simulink model "s_b4a4x32kf_nb"  (R2018a)
settings: Solver=VariableStepDiscrete  StartTime=0.0  StopTime=10000  RelTol=1e-3
undefined symbols (not defined in the file): fft_stages, n_bits_ants, n_bits_xengs
libraries: xbsIndex_r4 x21193, casper_library_misc x37, casper_library_scopes x13, casper_library_delays x8, xbsReplacements_r4 x6, xps_library x4
(part 162 of 274)

== system s_b4a4x32kf_nb/sys2/vacc/hmc_vacc/fifo_rd_cnt ==
  out_reg : Inport
  assert_reg : xbsIndex_r4/Assert  assert_type=on  type_source=Explicitly  gui_display_data_type=Fixed-point  arith_type=Unsigned  n_bits=32  bin_pt=0  preci_type=Single  exp_width=8  frac_width=24  assert_rate=off  rate_source=Explicitly  period=1  output_port=on  block_type=assert
      settings: SourceProductName=The database /home/jmanley/.matlab/R2018a/slblocks_master.db is locked, or a table in the database is locked. (database is locked)
  cast_gw : xbsIndex_r4/Convert  gui_display_data_type=Fixed-point  arith_type=Unsigned  n_bits=32  bin_pt=0  float_type=Single  exp_bits=8  fraction_bits=24  quantization=Truncate  overflow=Wrap  en=off  latency=1  pipeline=off  dbl_ovrd=off  block_type=convert
      settings: SourceProductName=The database /home/jmanley/.matlab/R2018a/slblocks_master.db is locked, or a table in the database is locked. (database is locked)
  io_delay : xbsIndex_r4/Delay  rst=off  infoeditControl=Selection of Reset will increase slice count due to use of real FFs and instead of SRLs  en=off  latency=0  reg_retiming=on  dbl_ovrd=off  block_type=delay
      settings: SourceProductName=The database /home/jmanley/.matlab/R2018a/slblocks_master.db is locked, or a table in the database is locked. (database is locked)
  reint1 : xbsIndex_r4/Reinterpret  force_arith_type=on  arith_type=Unsigned  force_bin_pt=on  bin_pt=0  block_type=reinterpret
      settings: SourceProductName=The database /home/jmanley/.matlab/R2018a/slblocks_master.db is locked, or a table in the database is locked. (database is locked)
  s_b4a4x32kf_nb_sys2_vacc_hmc_vacc_fifo_rd_cnt_user_data_in : xbsIndex_r4/Gateway Out  inherit_from_input=off  hdl_port=on  rows=1  columns=1  UseAsDAC=off  DACChannel='1'  interface=None  automatic_assignment=on  address_offset=hex2dec('00')  intf_name=''  intf_description=''  timing_constraint=None  locs_specified=off  LOCs={}  io_standard={}  block_type=gatewayout
      settings: SourceProductName=The database /home/jmanley/.matlab/R2018a/slblocks_master.db is locked, or a table in the database is locked. (database is locked)
  sim_out : Terminator
  wires:
  io_delay/1 -> cast_gw/1
  cast_gw/1 -> s_b4a4x32kf_nb_sys2_vacc_hmc_vacc_fifo_rd_cnt_user_data_in/1
  s_b4a4x32kf_nb_sys2_vacc_hmc_vacc_fifo_rd_cnt_user_data_in/1 -> sim_out/1
  out_reg/1 -> assert_reg/1
  assert_reg/1 -> reint1/1
  reint1/1 -> io_delay/1

== system s_b4a4x32kf_nb/sys2/vacc/hmc_vacc/fifo_status ==
  out_fetch_valid : Inport
  out_fetch_empty : Inport  Port=2
  out_fetch_full : Inport  Port=3
  out_fetch_afull : Inport  Port=4
  out_rst : Inport  Port=5
  out_fifo_rd_en : Inport  Port=6
  out_rb_en : Inport  Port=7
  out_out_ack : Inport  Port=8
  out_output_full : Inport  Port=9
  out_output_over : Inport  Port=10
  out_input_empty : Inport  Port=11
  out_input_over : Inport  Port=12
  out_output_empty : Inport  Port=13
  assert_fetch_afull : xbsIndex_r4/Assert  assert_type=on  type_source=Explicitly  gui_display_data_type=Boolean  arith_type=Boolean  n_bits=1  bin_pt=0  preci_type=Single  exp_width=8  frac_width=24  assert_rate=off  rate_source=Explicitly  period=1  output_port=on  block_type=assert
      settings: SourceProductName=The database /home/jmanley/.matlab/R2018a/slblocks_master.db is locked, or a table in the database is locked. (database is locked)
  assert_fetch_empty : xbsIndex_r4/Assert  assert_type=on  type_source=Explicitly  gui_display_data_type=Boolean  arith_type=Boolean  n_bits=1  bin_pt=0  preci_type=Single  exp_width=8  frac_width=24  assert_rate=off  rate_source=Explicitly  period=1  output_port=on  block_type=assert
      settings: SourceProductName=The database /home/jmanley/.matlab/R2018a/slblocks_master.db is locked, or a table in the database is locked. (database is locked)
  assert_fetch_full : xbsIndex_r4/Assert  assert_type=on  type_source=Explicitly  gui_display_data_type=Boolean  arith_type=Boolean  n_bits=1  bin_pt=0  preci_type=Single  exp_width=8  frac_width=24  assert_rate=off  rate_source=Explicitly  period=1  output_port=on  block_type=assert
      settings: SourceProductName=The database /home/jmanley/.matlab/R2018a/slblocks_master.db is locked, or a table in the database is locked. (database is locked)
  assert_fetch_valid : xbsIndex_r4/Assert  assert_type=on  type_source=Explicitly  gui_display_data_type=Boolean  arith_type=Boolean  n_bits=1  bin_pt=0  preci_type=Single  exp_width=8  frac_width=24  assert_rate=off  rate_source=Explicitly  period=1  output_port=on  block_type=assert
      settings: SourceProductName=The database /home/jmanley/.matlab/R2018a/slblocks_master.db is locked, or a table in the database is locked. (database is locked)
  assert_fifo_rd_en : xbsIndex_r4/Assert  assert_type=on  type_source=Explicitly  gui_display_data_type=Boolean  arith_type=Boolean  n_bits=1  bin_pt=0  preci_type=Single  exp_width=8  frac_width=24  assert_rate=off  rate_source=Explicitly  period=1  output_port=on  block_type=assert
      settings: SourceProductName=The database /home/jmanley/.matlab/R2018a/slblocks_master.db is locked, or a table in the database is locked. (database is locked)
  assert_input_empty : xbsIndex_r4/Assert  assert_type=on  type_source=Explicitly  gui_display_data_type=Boolean  arith_type=Boolean  n_bits=1  bin_pt=0  preci_type=Single  exp_width=8  frac_width=24  assert_rate=off  rate_source=Explicitly  period=1  output_port=on  block_type=assert
      settings: SourceProductName=The database /home/jmanley/.matlab/R2018a/slblocks_master.db is locked, or a table in the database is locked. (database is locked)
  assert_input_over : xbsIndex_r4/Assert  assert_type=on  type_source=Explicitly  gui_display_data_type=Boolean  arith_type=Boolean  n_bits=1  bin_pt=0  preci_type=Single  exp_width=8  frac_width=24  assert_rate=off  rate_source=Explicitly  period=1  output_port=on  block_type=assert
      settings: SourceProductName=The database /home/jmanley/.matlab/R2018a/slblocks_master.db is locked, or a table in the database is locked. (database is locked)
  assert_out_ack : xbsIndex_r4/Assert  assert_type=on  type_source=Explicitly  gui_display_data_type=Boolean  arith_type=Boolean  n_bits=1  bin_pt=0  preci_type=Single  exp_width=8  frac_width=24  assert_rate=off  rate_source=Explicitly  period=1  output_port=on  block_type=assert
      settings: SourceProductName=The database /home/jmanley/.matlab/R2018a/slblocks_master.db is locked, or a table in the database is locked. (database is locked)
  assert_output_empty : xbsIndex_r4/Assert  assert_type=on  type_source=Explicitly  gui_display_data_type=Boolean  arith_type=Boolean  n_bits=1  bin_pt=0  preci_type=Single  exp_width=8  frac_width=24  assert_rate=off  rate_source=Explicitly  period=1  output_port=on  block_type=assert
      settings: SourceProductName=The database /home/jmanley/.matlab/R2018a/slblocks_master.db is locked, or a table in the database is locked. (database is locked)
  assert_output_full : xbsIndex_r4/Assert  assert_type=on  type_source=Explicitly  gui_display_data_type=Boolean  arith_type=Boolean  n_bits=1  bin_pt=0  preci_type=Single  exp_width=8  frac_width=24  assert_rate=off  rate_source=Explicitly  period=1  output_port=on  block_type=assert
      settings: SourceProductName=The database /home/jmanley/.matlab/R2018a/slblocks_master.db is locked, or a table in the database is locked. (database is locked)
  assert_output_over : xbsIndex_r4/Assert  assert_type=on  type_source=Explicitly  gui_display_data_type=Boolean  arith_type=Boolean  n_bits=1  bin_pt=0  preci_type=Single  exp_width=8  frac_width=24  assert_rate=off  rate_source=Explicitly  period=1  output_port=on  block_type=assert
      settings: SourceProductName=The database /home/jmanley/.matlab/R2018a/slblocks_master.db is locked, or a table in the database is locked. (database is locked)
  assert_rb_en : xbsIndex_r4/Assert  assert_type=on  type_source=Explicitly  gui_display_data_type=Boolean  arith_type=Boolean  n_bits=1  bin_pt=0  preci_type=Single  exp_width=8  frac_width=24  assert_rate=off  rate_source=Explicitly  period=1  output_port=on  block_type=assert
      settings: SourceProductName=The database /home/jmanley/.matlab/R2018a/slblocks_master.db is locked, or a table in the database is locked. (database is locked)
  assert_rst : xbsIndex_r4/Assert  assert_type=on  type_source=Explicitly  gui_display_data_type=Boolean  arith_type=Boolean  n_bits=1  bin_pt=0  preci_type=Single  exp_width=8  frac_width=24  assert_rate=off  rate_source=Explicitly  period=1  output_port=on  block_type=assert
      settings: SourceProductName=The database /home/jmanley/.matlab/R2018a/slblocks_master.db is locked, or a table in the database is locked. (database is locked)
  cast_gw : xbsIndex_r4/Convert  gui_display_data_type=Fixed-point  arith_type=Unsigned  n_bits=32  bin_pt=0  float_type=Single  exp_bits=8  fraction_bits=24  quantization=Truncate  overflow=Wrap  en=off  latency=1  pipeline=off  dbl_ovrd=off  block_type=convert
      settings: SourceProductName=The database /home/jmanley/.matlab/R2018a/slblocks_master.db is locked, or a table in the database is locked. (database is locked)
  concatenate : xbsIndex_r4/Concat  num_inputs=13  dbl_ovrd=off  block_type=concat
      settings: SourceProductName=The database /home/jmanley/.matlab/R2018a/slblocks_master.db is locked, or a table in the database is locked. (database is locked)
  io_delay : xbsIndex_r4/Delay  rst=off  infoeditControl=Selection of Reset will increase slice count due to use of real FFs and instead of SRLs  en=off  latency=0  reg_retiming=on  dbl_ovrd=off  block_type=delay
      settings: SourceProductName=The database /home/jmanley/.matlab/R2018a/slblocks_master.db is locked, or a table in the database is locked. (database is locked)
  reint{1..13} (13 alike) : xbsIndex_r4/Reinterpret  force_arith_type=on  arith_type=Unsigned  force_bin_pt=on  bin_pt=0  block_type=reinterpret
      settings: SourceProductName=The database /home/jmanley/.matlab/R2018a/slblocks_master.db is locked, or a table in the database is locked. (database is locked)
  s_b4a4x32kf_nb_sys2_vacc_hmc_vacc_fifo_status_user_data_in : xbsIndex_r4/Gateway Out  inherit_from_input=off  hdl_port=on  rows=1  columns=1  UseAsDAC=off  DACChannel='1'  interface=None  automatic_assignment=on  address_offset=hex2dec('00')  intf_name=''  intf_description=''  timing_constraint=None  locs_specified=off  LOCs={}  io_standard={}  block_type=gatewayout
      settings: SourceProductName=The database /home/jmanley/.matlab/R2018a/slblocks_master.db is locked, or a table in the database is locked. (database is locked)
  sim_out : Terminator
  wires:
  concatenate/1 -> io_delay/1
  io_delay/1 -> cast_gw/1
  cast_gw/1 -> s_b4a4x32kf_nb_sys2_vacc_hmc_vacc_fifo_status_user_data_in/1
  s_b4a4x32kf_nb_sys2_vacc_hmc_vacc_fifo_status_user_data_in/1 -> sim_out/1
  out_fetch_valid/1 -> assert_fetch_valid/1
  assert_fetch_valid/1 -> reint1/1
  reint1/1 -> concatenate/1
  out_fetch_empty/1 -> assert_fetch_empty/1
  assert_fetch_empty/1 -> reint2/1
  reint2/1 -> concatenate/2
  out_fetch_full/1 -> assert_fetch_full/1
  assert_fetch_full/1 -> reint3/1
  reint3/1 -> concatenate/3
  out_fetch_afull/1 -> assert_fetch_afull/1
  assert_fetch_afull/1 -> reint4/1
  reint4/1 -> concatenate/4
  out_rst/1 -> assert_rst/1
  assert_rst/1 -> reint5/1
  reint5/1 -> concatenate/5
  out_fifo_rd_en/1 -> assert_fifo_rd_en/1
  assert_fifo_rd_en/1 -> reint6/1
  reint6/1 -> concatenate/6
  out_rb_en/1 -> assert_rb_en/1
  assert_rb_en/1 -> reint7/1
  reint7/1 -> concatenate/7
  out_out_ack/1 -> assert_out_ack/1
  assert_out_ack/1 -> reint8/1
  reint8/1 -> concatenate/8
  out_output_full/1 -> assert_output_full/1
  assert_output_full/1 -> reint9/1
  reint9/1 -> concatenate/9
  out_output_over/1 -> assert_output_over/1
  assert_output_over/1 -> reint10/1
  reint10/1 -> concatenate/10
  out_input_empty/1 -> assert_input_empty/1
  assert_input_empty/1 -> reint11/1
  reint11/1 -> concatenate/11
  out_input_over/1 -> assert_input_over/1
  assert_input_over/1 -> reint12/1
  reint12/1 -> concatenate/12
  out_output_empty/1 -> assert_output_empty/1
  assert_output_empty/1 -> reint13/1
  reint13/1 -> concatenate/13

== system s_b4a4x32kf_nb/sys2/vacc/hmc_vacc/fifo_wr_cnt ==
  out_reg : Inport
  assert_reg : xbsIndex_r4/Assert  assert_type=on  type_source=Explicitly  gui_display_data_type=Fixed-point  arith_type=Unsigned  n_bits=32  bin_pt=0  preci_type=Single  exp_width=8  frac_width=24  assert_rate=off  rate_source=Explicitly  period=1  output_port=on  block_type=assert
      settings: SourceProductName=The database /home/jmanley/.matlab/R2018a/slblocks_master.db is locked, or a table in the database is locked. (database is locked)
  cast_gw : xbsIndex_r4/Convert  gui_display_data_type=Fixed-point  arith_type=Unsigned  n_bits=32  bin_pt=0  float_type=Single  exp_bits=8  fraction_bits=24  quantization=Truncate  overflow=Wrap  en=off  latency=1  pipeline=off  dbl_ovrd=off  block_type=convert
      settings: SourceProductName=The database /home/jmanley/.matlab/R2018a/slblocks_master.db is locked, or a table in the database is locked. (database is locked)
  io_delay : xbsIndex_r4/Delay  rst=off  infoeditControl=Selection of Reset will increase slice count due to use of real FFs and instead of SRLs  en=off  latency=0  reg_retiming=on  dbl_ovrd=off  block_type=delay
      settings: SourceProductName=The database /home/jmanley/.matlab/R2018a/slblocks_master.db is locked, or a table in the database is locked. (database is locked)
  reint1 : xbsIndex_r4/Reinterpret  force_arith_type=on  arith_type=Unsigned  force_bin_pt=on  bin_pt=0  block_type=reinterpret
      settings: SourceProductName=The database /home/jmanley/.matlab/R2018a/slblocks_master.db is locked, or a table in the database is locked. (database is locked)
  s_b4a4x32kf_nb_sys2_vacc_hmc_vacc_fifo_wr_cnt_user_data_in : xbsIndex_r4/Gateway Out  inherit_from_input=off  hdl_port=on  rows=1  columns=1  UseAsDAC=off  DACChannel='1'  interface=None  automatic_assignment=on  address_offset=hex2dec('00')  intf_name=''  intf_description=''  timing_constraint=None  locs_specified=off  LOCs={}  io_standard={}  block_type=gatewayout
      settings: SourceProductName=The database /home/jmanley/.matlab/R2018a/slblocks_master.db is locked, or a table in the database is locked. (database is locked)
  sim_out : Terminator
  wires:
  io_delay/1 -> cast_gw/1
  cast_gw/1 -> s_b4a4x32kf_nb_sys2_vacc_hmc_vacc_fifo_wr_cnt_user_data_in/1
  s_b4a4x32kf_nb_sys2_vacc_hmc_vacc_fifo_wr_cnt_user_data_in/1 -> sim_out/1
  out_reg/1 -> assert_reg/1
  assert_reg/1 -> reint1/1
  reint1/1 -> io_delay/1

== system s_b4a4x32kf_nb/sys2/vacc/hmc_vacc/half_sel ==
  In1 : Inport
  Concat1 : xbsIndex_r4/Concat  num_inputs=3  dbl_ovrd=off  block_type=concat
      settings: SourceProductName=The database /home/jmanley/.matlab/R2018a/slblocks_master.db is locked, or a table in the database is locked. (database is locked)  block_version=10.1.3
  Constant3 : xbsIndex_r4/Constant  const=link  gui_display_data_type=Fixed-point  arith_type=Unsigned  n_bits=1  bin_pt=0  preci_type=Single  exp_width=8  frac_width=24  explicit_period=on  period=1  equ=P=C  opselect=C  inp2=PCIN>>17  opr=+  inp1=P  carry=CIN  dbl_ovrd=off  block_type=constant
      settings: SourceProductName=The database /home/jmanley/.matlab/R2018a/slblocks_master.db is locked, or a table in the database is locked. (database is locked)
  Slice1 : xbsIndex_r4/Slice  nbits=2  boolean_output=off  mode=Lower Bit Location + Width  bit1=96  base1=MSB of Input  bit0=0  base0=LSB of Input  dbl_ovrd=off  block_type=slice
      settings: SourceProductName=The database /home/jmanley/.matlab/R2018a/slblocks_master.db is locked, or a table in the database is locked. (database is locked)  block_version=9.2.01
  Slice5 : xbsIndex_r4/Slice  nbits=23  boolean_output=off  mode=Two Bit Locations  bit1=0  base1=MSB of Input  bit0=2  base0=LSB of Input  dbl_ovrd=off  block_type=slice
      settings: SourceProductName=The database /home/jmanley/.matlab/R2018a/slblocks_master.db is locked, or a table in the database is locked. (database is locked)  block_version=9.2.01
  Out1 : Outport
  wires:
  In1/1 -> Slice1/1, Slice5/1
  Slice5/1 -> Concat1/1
  Constant3/1 -> Concat1/2
  Slice1/1 -> Concat1/3
  Concat1/1 -> Out1/1

== system s_b4a4x32kf_nb/sys2/vacc/hmc_vacc/half_sel1 ==
  In1 : Inport
  Concat1 : xbsIndex_r4/Concat  num_inputs=3  dbl_ovrd=off  block_type=concat
      settings: SourceProductName=The database /home/jmanley/.matlab/R2018a/slblocks_master.db is locked, or a table in the database is locked. (database is locked)  block_version=10.1.3
  Constant3 : xbsIndex_r4/Constant  const=link  gui_display_data_type=Fixed-point  arith_type=Unsigned  n_bits=1  bin_pt=0  preci_type=Single  exp_width=8  frac_width=24  explicit_period=on  period=1  equ=P=C  opselect=C  inp2=PCIN>>17  opr=+  inp1=P  carry=CIN  dbl_ovrd=off  block_type=constant
      settings: SourceProductName=The database /home/jmanley/.matlab/R2018a/slblocks_master.db is locked, or a table in the database is locked. (database is locked)
  Slice1 : xbsIndex_r4/Slice  nbits=2  boolean_output=off  mode=Lower Bit Location + Width  bit1=96  base1=MSB of Input  bit0=0  base0=LSB of Input  dbl_ovrd=off  block_type=slice
      settings: SourceProductName=The database /home/jmanley/.matlab/R2018a/slblocks_master.db is locked, or a table in the database is locked. (database is locked)  block_version=9.2.01
  Slice5 : xbsIndex_r4/Slice  nbits=23  boolean_output=off  mode=Two Bit Locations  bit1=0  base1=MSB of Input  bit0=2  base0=LSB of Input  dbl_ovrd=off  block_type=slice
      settings: SourceProductName=The database /home/jmanley/.matlab/R2018a/slblocks_master.db is locked, or a table in the database is locked. (database is locked)  block_version=9.2.01
  Out1 : Outport
  wires:
  In1/1 -> Slice1/1, Slice5/1
  Slice5/1 -> Concat1/1
  Constant3/1 -> Concat1/2
  Slice1/1 -> Concat1/3
  Concat1/1 -> Out1/1

== system s_b4a4x32kf_nb/sys2/vacc/hmc_vacc/half_sel2 ==
  In1 : Inport
  Concat1 : xbsIndex_r4/Concat  num_inputs=3  dbl_ovrd=off  block_type=concat
      settings: SourceProductName=The database /home/jmanley/.matlab/R2018a/slblocks_master.db is locked, or a table in the database is locked. (database is locked)  block_version=10.1.3
  Constant3 : xbsIndex_r4/Constant  const=link  gui_display_data_type=Fixed-point  arith_type=Unsigned  n_bits=1  bin_pt=0  preci_type=Single  exp_width=8  frac_width=24  explicit_period=on  period=1  equ=P=C  opselect=C  inp2=PCIN>>17  opr=+  inp1=P  carry=CIN  dbl_ovrd=off  block_type=constant
      settings: SourceProductName=The database /home/jmanley/.matlab/R2018a/slblocks_master.db is locked, or a table in the database is locked. (database is locked)
  Slice1 : xbsIndex_r4/Slice  nbits=2  boolean_output=off  mode=Lower Bit Location + Width  bit1=96  base1=MSB of Input  bit0=0  base0=LSB of Input  dbl_ovrd=off  block_type=slice
      settings: SourceProductName=The database /home/jmanley/.matlab/R2018a/slblocks_master.db is locked, or a table in the database is locked. (database is locked)  block_version=9.2.01
  Slice5 : xbsIndex_r4/Slice  nbits=23  boolean_output=off  mode=Two Bit Locations  bit1=0  base1=MSB of Input  bit0=2  base0=LSB of Input  dbl_ovrd=off  block_type=slice
      settings: SourceProductName=The database /home/jmanley/.matlab/R2018a/slblocks_master.db is locked, or a table in the database is locked. (database is locked)  block_version=9.2.01
  Out1 : Outport
  wires:
  In1/1 -> Slice1/1, Slice5/1
  Slice5/1 -> Concat1/1
  Constant3/1 -> Concat1/2
  Slice1/1 -> Concat1/3
  Concat1/1 -> Out1/1

== system s_b4a4x32kf_nb/sys2/vacc/hmc_vacc/half_sel3 ==
  In1 : Inport
  Concat1 : xbsIndex_r4/Concat  num_inputs=3  dbl_ovrd=off  block_type=concat
      settings: SourceProductName=The database /home/jmanley/.matlab/R2018a/slblocks_master.db is locked, or a table in the database is locked. (database is locked)  block_version=10.1.3
  Constant3 : xbsIndex_r4/Constant  const=link  gui_display_data_type=Fixed-point  arith_type=Unsigned  n_bits=1  bin_pt=0  preci_type=Single  exp_width=8  frac_width=24  explicit_period=on  period=1  equ=P=C  opselect=C  inp2=PCIN>>17  opr=+  inp1=P  carry=CIN  dbl_ovrd=off  block_type=constant
      settings: SourceProductName=The database /home/jmanley/.matlab/R2018a/slblocks_master.db is locked, or a table in the database is locked. (database is locked)
  Slice1 : xbsIndex_r4/Slice  nbits=2  boolean_output=off  mode=Lower Bit Location + Width  bit1=96  base1=MSB of Input  bit0=0  base0=LSB of Input  dbl_ovrd=off  block_type=slice
      settings: SourceProductName=The database /home/jmanley/.matlab/R2018a/slblocks_master.db is locked, or a table in the database is locked. (database is locked)  block_version=9.2.01
  Slice5 : xbsIndex_r4/Slice  nbits=23  boolean_output=off  mode=Two Bit Locations  bit1=0  base1=MSB of Input  bit0=2  base0=LSB of Input  dbl_ovrd=off  block_type=slice
      settings: SourceProductName=The database /home/jmanley/.matlab/R2018a/slblocks_master.db is locked, or a table in the database is locked. (database is locked)  block_version=9.2.01
  Out1 : Outport
  wires:
  Concat1/1 -> Out1/1
  Slice1/1 -> Concat1/3
  Constant3/1 -> Concat1/2
  Slice5/1 -> Concat1/1
  In1/1 -> Slice5/1, Slice1/1

== system s_b4a4x32kf_nb/sys2/vacc/hmc_vacc/hmc_out_cnt ==
  out_reg : Inport
  assert_reg : xbsIndex_r4/Assert  assert_type=on  type_source=Explicitly  gui_display_data_type=Fixed-point  arith_type=Unsigned  n_bits=32  bin_pt=0  preci_type=Single  exp_width=8  frac_width=24  assert_rate=off  rate_source=Explicitly  period=1  output_port=on  block_type=assert
      settings: SourceProductName=The database /home/jmanley/.matlab/R2018a/slblocks_master.db is locked, or a table in the database is locked. (database is locked)
  cast_gw : xbsIndex_r4/Convert  gui_display_data_type=Fixed-point  arith_type=Unsigned  n_bits=32  bin_pt=0  float_type=Single  exp_bits=8  fraction_bits=24  quantization=Truncate  overflow=Wrap  en=off  latency=1  pipeline=off  dbl_ovrd=off  block_type=convert
      settings: SourceProductName=The database /home/jmanley/.matlab/R2018a/slblocks_master.db is locked, or a table in the database is locked. (database is locked)
  io_delay : xbsIndex_r4/Delay  rst=off  infoeditControl=Selection of Reset will increase slice count due to use of real FFs and instead of SRLs  en=off  latency=0  reg_retiming=on  dbl_ovrd=off  block_type=delay
      settings: SourceProductName=The database /home/jmanley/.matlab/R2018a/slblocks_master.db is locked, or a table in the database is locked. (database is locked)
  reint1 : xbsIndex_r4/Reinterpret  force_arith_type=on  arith_type=Unsigned  force_bin_pt=on  bin_pt=0  block_type=reinterpret
      settings: SourceProductName=The database /home/jmanley/.matlab/R2018a/slblocks_master.db is locked, or a table in the database is locked. (database is locked)
  s_b4a4x32kf_nb_sys2_vacc_hmc_vacc_hmc_out_cnt_user_data_in : xbsIndex_r4/Gateway Out  inherit_from_input=off  hdl_port=on  rows=1  columns=1  UseAsDAC=off  DACChannel='1'  interface=None  automatic_assignment=on  address_offset=hex2dec('00')  intf_name=''  intf_description=''  timing_constraint=None  locs_specified=off  LOCs={}  io_standard={}  block_type=gatewayout
      settings: SourceProductName=The database /home/jmanley/.matlab/R2018a/slblocks_master.db is locked, or a table in the database is locked. (database is locked)
  sim_out : Terminator
  wires:
  io_delay/1 -> cast_gw/1
  cast_gw/1 -> s_b4a4x32kf_nb_sys2_vacc_hmc_vacc_hmc_out_cnt_user_data_in/1
  s_b4a4x32kf_nb_sys2_vacc_hmc_vacc_hmc_out_cnt_user_data_in/1 -> sim_out/1
  out_reg/1 -> assert_reg/1
  assert_reg/1 -> reint1/1
  reint1/1 -> io_delay/1

== system s_b4a4x32kf_nb/sys2/vacc/hmc_vacc/hmc_rd_cnt ==
  out_reg : Inport
  assert_reg : xbsIndex_r4/Assert  assert_type=on  type_source=Explicitly  gui_display_data_type=Fixed-point  arith_type=Unsigned  n_bits=32  bin_pt=0  preci_type=Single  exp_width=8  frac_width=24  assert_rate=off  rate_source=Explicitly  period=1  output_port=on  block_type=assert
      settings: SourceProductName=The database /home/jmanley/.matlab/R2018a/slblocks_master.db is locked, or a table in the database is locked. (database is locked)
  cast_gw : xbsIndex_r4/Convert  gui_display_data_type=Fixed-point  arith_type=Unsigned  n_bits=32  bin_pt=0  float_type=Single  exp_bits=8  fraction_bits=24  quantization=Truncate  overflow=Wrap  en=off  latency=1  pipeline=off  dbl_ovrd=off  block_type=convert
      settings: SourceProductName=The database /home/jmanley/.matlab/R2018a/slblocks_master.db is locked, or a table in the database is locked. (database is locked)
  io_delay : xbsIndex_r4/Delay  rst=off  infoeditControl=Selection of Reset will increase slice count due to use of real FFs and instead of SRLs  en=off  latency=0  reg_retiming=on  dbl_ovrd=off  block_type=delay
      settings: SourceProductName=The database /home/jmanley/.matlab/R2018a/slblocks_master.db is locked, or a table in the database is locked. (database is locked)
  reint1 : xbsIndex_r4/Reinterpret  force_arith_type=on  arith_type=Unsigned  force_bin_pt=on  bin_pt=0  block_type=reinterpret
      settings: SourceProductName=The database /home/jmanley/.matlab/R2018a/slblocks_master.db is locked, or a table in the database is locked. (database is locked)
  s_b4a4x32kf_nb_sys2_vacc_hmc_vacc_hmc_rd_cnt_user_data_in : xbsIndex_r4/Gateway Out  inherit_from_input=off  hdl_port=on  rows=1  columns=1  UseAsDAC=off  DACChannel='1'  interface=None  automatic_assignment=on  address_offset=hex2dec('00')  intf_name=''  intf_description=''  timing_constraint=None  locs_specified=off  LOCs={}  io_standard={}  block_type=gatewayout
      settings: SourceProductName=The database /home/jmanley/.matlab/R2018a/slblocks_master.db is locked, or a table in the database is locked. (database is locked)
  sim_out : Terminator
  wires:
  io_delay/1 -> cast_gw/1
  cast_gw/1 -> s_b4a4x32kf_nb_sys2_vacc_hmc_vacc_hmc_rd_cnt_user_data_in/1
  s_b4a4x32kf_nb_sys2_vacc_hmc_vacc_hmc_rd_cnt_user_data_in/1 -> sim_out/1
  out_reg/1 -> assert_reg/1
  assert_reg/1 -> reint1/1
  reint1/1 -> io_delay/1

== system s_b4a4x32kf_nb/sys2/vacc/hmc_vacc/hmc_reord ==
  note: delay rst a bit longer than needed,
      | just in case.
      | HMC won't output valid data for a
      | while after the VACC comes out of reset
  note: clear the valid
      | entries on reset
  rst : Inport
  data_in : Inport  Port=2
  valid_in : Inport  Port=3
  tag_in : Inport  Port=4
  Concat : xbsIndex_r4/Concat  num_inputs=3  dbl_ovrd=off  block_type=concat
      settings: SourceProductName=The database /home/jmanley/.matlab/R2018a/slblocks_master.db is locked, or a table in the database is locked. (database is locked)
  Constant2 : xbsIndex_r4/Constant  const=0  gui_display_data_type=Fixed-point  arith_type=Unsigned  n_bits=266  bin_pt=0  preci_type=Single  exp_width=8  frac_width=24  explicit_period=on  period=1  equ=P=C  opselect=C  inp2=PCIN>>17  opr=+  inp1=P  carry=CIN  dbl_ovrd=off  block_type=constant
      settings: SourceProductName=The database /home/jmanley/.matlab/R2018a/slblocks_master.db is locked, or a table in the database is locked. (database is locked)
  Constant3 : xbsIndex_r4/Constant  const=1  gui_display_data_type=Fixed-point  arith_type=Unsigned  n_bits=1  bin_pt=0  preci_type=Single  exp_width=8  frac_width=24  explicit_period=on  period=1  equ=P=C  opselect=C  inp2=PCIN>>17  opr=+  inp1=P  carry=CIN  dbl_ovrd=off  block_type=constant
      settings: SourceProductName=The database /home/jmanley/.matlab/R2018a/slblocks_master.db is locked, or a table in the database is locked. (database is locked)
  Convert : xbsIndex_r4/Convert  gui_display_data_type=Boolean  arith_type=Boolean  n_bits=1  bin_pt=0  float_type=Single  exp_bits=8  fraction_bits=24  quantization=Truncate  overflow=Wrap  en=off  latency=0  pipeline=off  dbl_ovrd=off  block_type=convert
      settings: SourceProductName=The database /home/jmanley/.matlab/R2018a/slblocks_master.db is locked, or a table in the database is locked. (database is locked)
  Delay1 : xbsIndex_r4/Delay  rst=off  infoeditControl=Selection of Reset will increase slice count due to use of real FFs and instead of SRLs  en=off  latency=2  reg_retiming=off  dbl_ovrd=off  block_type=delay
      settings: SourceProductName=The database /home/jmanley/.matlab/R2018a/slblocks_master.db is locked, or a table in the database is locked. (database is locked)  infoedit=Hardware notes: A delay line is a chain, each link of which is an SRL16 or SRL32 followed by a flip-flop.
  Delay6 : xbsIndex_r4/Delay  rst=off  infoeditControl=Selection of Reset will increase slice count due to use of real FFs and instead of SRLs  en=off  latency=1  reg_retiming=off  dbl_ovrd=off  block_type=delay
      settings: SourceProductName=The database /home/jmanley/.matlab/R2018a/slblocks_master.db is locked, or a table in the database is locked. (database is locked)  infoedit=Hardware notes: A delay line is a chain, each link of which is an SRL16 or SRL32 followed by a flip-flop.
  Delay7 : xbsIndex_r4/Delay  rst=off  infoeditControl=Selection of Reset will increase slice count due to use of real FFs and instead of SRLs  en=off  latency=1  reg_retiming=off  dbl_ovrd=off  block_type=delay
      settings: SourceProductName=The database /home/jmanley/.matlab/R2018a/slblocks_master.db is locked, or a table in the database is locked. (database is locked)  infoedit=Hardware notes: A delay line is a chain, each link of which is an SRL16 or SRL32 followed by a flip-flop.
  Delay8 : xbsIndex_r4/Delay  rst=off  infoeditControl=Selection of Reset will increase slice count due to use of real FFs and instead of SRLs  en=off  latency=1  reg_retiming=off  dbl_ovrd=off  block_type=delay
      settings: SourceProductName=The database /home/jmanley/.matlab/R2018a/slblocks_master.db is locked, or a table in the database is locked. (database is locked)  infoedit=Hardware notes: A delay line is a chain, each link of which is an SRL16 or SRL32 followed by a flip-flop.
  Delay9 : xbsIndex_r4/Delay  rst=off  infoeditControl=Selection of Reset will increase slice count due to use of real FFs and instead of SRLs  en=off  latency=2  reg_retiming=off  dbl_ovrd=off  block_type=delay
      settings: SourceProductName=The database /home/jmanley/.matlab/R2018a/slblocks_master.db is locked, or a table in the database is locked. (database is locked)  infoedit=Hardware notes: A delay line is a chain, each link of which is an SRL16 or SRL32 followed by a flip-flop.
  Inverter : xbsIndex_r4/Inverter  en=off  latency=0  dbl_ovrd=off  block_type=inv
      settings: SourceProductName=The database /home/jmanley/.matlab/R2018a/slblocks_master.db is locked, or a table in the database is locked. (database is locked)
  Inverter1 : xbsIndex_r4/Inverter  en=off  latency=0  dbl_ovrd=off  block_type=inv
      settings: SourceProductName=The database /home/jmanley/.matlab/R2018a/slblocks_master.db is locked, or a table in the database is locked. (database is locked)
  Logical : xbsIndex_r4/Logical  logical_function=AND  inputs=2  en=off  latency=0  precision=Full  arith_type=Unsigned  n_bits=16  bin_pt=0  align_bp=on  dbl_ovrd=off  block_type=logical
      settings: SourceProductName=The database /home/jmanley/.matlab/R2018a/slblocks_master.db is locked, or a table in the database is locked. (database is locked)
  Logical1 : xbsIndex_r4/Logical  logical_function=OR  inputs=2  en=off  latency=0  precision=Full  arith_type=Unsigned  n_bits=16  bin_pt=0  align_bp=on  dbl_ovrd=off  block_type=logical
      settings: SourceProductName=The database /home/jmanley/.matlab/R2018a/slblocks_master.db is locked, or a table in the database is locked. (database is locked)
  Logical2 : xbsIndex_r4/Logical  logical_function=OR  inputs=2  en=off  latency=0  precision=Full  arith_type=Unsigned  n_bits=16  bin_pt=0  align_bp=on  dbl_ovrd=off  block_type=logical
      settings: SourceProductName=The database /home/jmanley/.matlab/R2018a/slblocks_master.db is locked, or a table in the database is locked. (database is locked)
  Logical3 : xbsIndex_r4/Logical  logical_function=AND  inputs=2  en=off  latency=0  precision=Full  arith_type=Unsigned  n_bits=16  bin_pt=0  align_bp=on  dbl_ovrd=off  block_type=logical
      settings: SourceProductName=The database /home/jmanley/.matlab/R2018a/slblocks_master.db is locked, or a table in the database is locked. (database is locked)
  Slice1 : xbsIndex_r4/Slice  nbits=256  boolean_output=off  mode=Lower Bit Location + Width  bit1=0  base1=MSB of Input  bit0=9  base0=LSB of Input  dbl_ovrd=off  block_type=slice
      settings: SourceProductName=The database /home/jmanley/.matlab/R2018a/slblocks_master.db is locked, or a table in the database is locked. (database is locked)  block_version=9.2.01
  Slice11 : xbsIndex_r4/Slice  nbits=9  boolean_output=off  mode=Lower Bit Location + Width  bit1=-1  base1=MSB of Input  bit0=0  base0=LSB of Input  dbl_ovrd=off  block_type=slice
      settings: SourceProductName=The database /home/jmanley/.matlab/R2018a/slblocks_master.db is locked, or a table in the database is locked. (database is locked)  block_version=9.2.01
  Slice2 : xbsIndex_r4/Slice  nbits=1  boolean_output=off  mode=Upper Bit Location + Width  bit1=0  base1=MSB of Input  bit0=0  base0=LSB of Input  dbl_ovrd=off  block_type=slice
      settings: SourceProductName=The database /home/jmanley/.matlab/R2018a/slblocks_master.db is locked, or a table in the database is locked. (database is locked)  block_version=9.2.01
  Slice3 : xbsIndex_r4/Slice  nbits=9  boolean_output=off  mode=Lower Bit Location + Width  bit1=-1  base1=MSB of Input  bit0=0  base0=LSB of Input  dbl_ovrd=off  block_type=slice
      settings: SourceProductName=The database /home/jmanley/.matlab/R2018a/slblocks_master.db is locked, or a table in the database is locked. (database is locked)  block_version=9.2.01
  Slice4 : xbsIndex_r4/Slice  nbits=9  boolean_output=off  mode=Lower Bit Location + Width  bit1=-1  base1=MSB of Input  bit0=0  base0=LSB of Input  dbl_ovrd=off  block_type=slice
      settings: SourceProductName=The database /home/jmanley/.matlab/R2018a/slblocks_master.db is locked, or a table in the database is locked. (database is locked)  block_version=9.2.01
  Slice5 : xbsIndex_r4/Slice  nbits=256  boolean_output=off  mode=Lower Bit Location + Width  bit1=-1  base1=MSB of Input  bit0=0  base0=LSB of Input  dbl_ovrd=off  block_type=slice
      settings: SourceProductName=The database /home/jmanley/.matlab/R2018a/slblocks_master.db is locked, or a table in the database is locked. (database is locked)  block_version=9.2.01
  dpr : xbsIndex_r4/Dual Port RAM  depth=512  initVector=0  distributed_mem=Block RAM  init_a=0  init_b=0  rst_a=off  rst_b=off  en_a=off  en_b=off  latency=2  write_mode_A=Read Before Write  write_mode_B=Read Before Write  optimize=Area  dbl_ovrd=off  block_type=dpram
      settings: SourceProductName=The database /home/jmanley/.matlab/R2018a/slblocks_master.db is locked, or a table in the database is locked. (database is locked)
  edge_detect2 : Subsystem  mask(edge_detect){edge=Falling, polarity=Active High, x_in=[0 0.08 0.08 0.16 0.16 0.24 0.24 0.32 0.32 0.4], y_in=[-1 -1  1  1  1  1  1  1  1  1], x_out=[0.6 0.68 0.68 0.76 0.76 0.84 0.84 0.92 0.92 1], y_out=[-1 -1  1  1 -1 -1 -1 -1 -1 -1]}
      mask prompts: edge "Edge Type"; polarity "Output Polarity"; x_in "Input X Positions"; y_in "Input Y Positions"; x_out "Output X Positions"; y_out "Output Y Positions"
      mask help: Output is active for one-cycle after each edge of the specified type (i.e. rising, falling or both).
      mask init: same as s_b4a4x32kf_nb/edge_detect
      settings: AttributesFormatString=|
      | falling edges
      | active high
      mask Help: Output is active for one-cycle after each edge of the specified type (i.e. rising, falling, or both).  Latency is zero.
      mask TypeOptions edge: Rising | Falling | Both
      mask TypeOptions polarity: Active High | Active Low
      mask Display:
      | plot(x_in_num,0.5+y_in_num*0.2);
      | plot(x_out_num,0.5+y_out_num*0.2);
  max_hold : Subsystem
  rd_index : xbsIndex_r4/Counter  cnt_type=Free Running  cnt_to=1  operation=Up  start_count=0  cnt_by_val=1  arith_type=Unsigned  n_bits=9  bin_pt=0  load_pin=off  rst=on  en=on  explicit_period=on  period=1  use_behavioral_HDL=off  implementation=Fabric  use_rpm=off  dbl_ovrd=off  block_type=counter
      settings: SourceProductName=The database /home/jmanley/.matlab/R2018a/slblocks_master.db is locked, or a table in the database is locked. (database is locked)
  run_like_the_wind : Subsystem  mask{window_size=250}
      mask prompts: window_size "randomness gap (words)"
  stutter : Subsystem  mask{latency=2}
      mask prompts: latency "BRAM latency"
  data_out : Outport
  valid_out : Outport  Port=2
  tag_out : Outport  Port=3
  err : Outport  Port=4
  wires:
  valid_in/1 -> [valid_in]
  tag_in/1 -> [tag_in], Slice3/1, Slice11/1
  Slice5/1 -> Concat/2
  data_in/1 -> Slice5/1
  Constant2/1 -> dpr/5
  dpr/2 -> Slice4/1, Slice2/1, Slice1/1
  rd_index/1 -> [rd_idx]
  Slice1/1 -> data_out/1
  Constant3/1 -> Concat/1
  Concat/1 -> dpr/2
  Slice2/1 -> Convert/1
  run_like_the_wind/1(rd_en) -> [run]
  Slice11/1 -> dpr/1, Delay6/1
  Convert/1 -> [mem_valid]
  Delay1/1 -> [valid_out], valid_out/1
  Logical2/1 -> Logical3/1, Logical1/1
  stutter/1(rd) -> [stutter]
  Slice3/1 -> Concat/3
  Slice4/1 -> tag_out/1
  max_hold/1(max) -> [max]
  rst/1 -> Delay7/1
  [rst] -> max_hold/3(rst)
  Delay7/1 -> [rst]
  Delay6/1 -> max_hold/1(value)
  Delay8/1 -> max_hold/2(valid)
  [valid_in] -> Delay8/1
  [valid_in] -> dpr/3
  [max] -> run_like_the_wind/1(max)
  [rd_idx] -> dpr/4
  [rd_idx] -> run_like_the_wind/2(rd_idx)
  [run] -> Logical2/1
  [stutter] -> Logical2/2
  [mem_valid] -> stutter/1(valid_mem)
  Logical/1 -> err/1
  [mem_valid] -> Inverter/1
  [valid_out] -> Logical/1
  Inverter/1 -> Logical/2
  [rst] -> edge_detect2/1(in)
  edge_detect2/1(out) -> rd_index/1
  Logical1/1 -> stutter/2(read_en), dpr/6, rd_index/2
  [rst] -> Logical1/2
  Inverter1/1 -> Logical3/2
  Logical3/1 -> Delay1/1
  [rst] -> Delay9/1
  Delay9/1 -> Inverter1/1

== system s_b4a4x32kf_nb/sys2/vacc/hmc_vacc/hmc_wr_cnt ==
  out_reg : Inport
  assert_reg : xbsIndex_r4/Assert  assert_type=on  type_source=Explicitly  gui_display_data_type=Fixed-point  arith_type=Unsigned  n_bits=32  bin_pt=0  preci_type=Single  exp_width=8  frac_width=24  assert_rate=off  rate_source=Explicitly  period=1  output_port=on  block_type=assert
      settings: SourceProductName=The database /home/jmanley/.matlab/R2018a/slblocks_master.db is locked, or a table in the database is locked. (database is locked)
  cast_gw : xbsIndex_r4/Convert  gui_display_data_type=Fixed-point  arith_type=Unsigned  n_bits=32  bin_pt=0  float_type=Single  exp_bits=8  fraction_bits=24  quantization=Truncate  overflow=Wrap  en=off  latency=1  pipeline=off  dbl_ovrd=off  block_type=convert
      settings: SourceProductName=The database /home/jmanley/.matlab/R2018a/slblocks_master.db is locked, or a table in the database is locked. (database is locked)
  io_delay : xbsIndex_r4/Delay  rst=off  infoeditControl=Selection of Reset will increase slice count due to use of real FFs and instead of SRLs  en=off  latency=0  reg_retiming=on  dbl_ovrd=off  block_type=delay
      settings: SourceProductName=The database /home/jmanley/.matlab/R2018a/slblocks_master.db is locked, or a table in the database is locked. (database is locked)
  reint1 : xbsIndex_r4/Reinterpret  force_arith_type=on  arith_type=Unsigned  force_bin_pt=on  bin_pt=0  block_type=reinterpret
      settings: SourceProductName=The database /home/jmanley/.matlab/R2018a/slblocks_master.db is locked, or a table in the database is locked. (database is locked)
  s_b4a4x32kf_nb_sys2_vacc_hmc_vacc_hmc_wr_cnt_user_data_in : xbsIndex_r4/Gateway Out  inherit_from_input=off  hdl_port=on  rows=1  columns=1  UseAsDAC=off  DACChannel='1'  interface=None  automatic_assignment=on  address_offset=hex2dec('00')  intf_name=''  intf_description=''  timing_constraint=None  locs_specified=off  LOCs={}  io_standard={}  block_type=gatewayout
      settings: SourceProductName=The database /home/jmanley/.matlab/R2018a/slblocks_master.db is locked, or a table in the database is locked. (database is locked)
  sim_out : Terminator
  wires:
  io_delay/1 -> cast_gw/1
  cast_gw/1 -> s_b4a4x32kf_nb_sys2_vacc_hmc_vacc_hmc_wr_cnt_user_data_in/1
  s_b4a4x32kf_nb_sys2_vacc_hmc_vacc_hmc_wr_cnt_user_data_in/1 -> sim_out/1
  out_reg/1 -> assert_reg/1
  assert_reg/1 -> reint1/1
  reint1/1 -> io_delay/1

== system s_b4a4x32kf_nb/sys2/vacc/hmc_vacc/miss_data_cnt ==
  out_reg : Inport
  assert_reg : xbsIndex_r4/Assert  assert_type=on  type_source=Explicitly  gui_display_data_type=Fixed-point  arith_type=Unsigned  n_bits=32  bin_pt=0  preci_type=Single  exp_width=8  frac_width=24  assert_rate=off  rate_source=Explicitly  period=1  output_port=on  block_type=assert
      settings: SourceProductName=The database /home/jmanley/.matlab/R2018a/slblocks_master.db is locked, or a table in the database is locked. (database is locked)
  cast_gw : xbsIndex_r4/Convert  gui_display_data_type=Fixed-point  arith_type=Unsigned  n_bits=32  bin_pt=0  float_type=Single  exp_bits=8  fraction_bits=24  quantization=Truncate  overflow=Wrap  en=off  latency=1  pipeline=off  dbl_ovrd=off  block_type=convert
      settings: SourceProductName=The database /home/jmanley/.matlab/R2018a/slblocks_master.db is locked, or a table in the database is locked. (database is locked)
  io_delay : xbsIndex_r4/Delay  rst=off  infoeditControl=Selection of Reset will increase slice count due to use of real FFs and instead of SRLs  en=off  latency=0  reg_retiming=on  dbl_ovrd=off  block_type=delay
      settings: SourceProductName=The database /home/jmanley/.matlab/R2018a/slblocks_master.db is locked, or a table in the database is locked. (database is locked)
  reint1 : xbsIndex_r4/Reinterpret  force_arith_type=on  arith_type=Unsigned  force_bin_pt=on  bin_pt=0  block_type=reinterpret
      settings: SourceProductName=The database /home/jmanley/.matlab/R2018a/slblocks_master.db is locked, or a table in the database is locked. (database is locked)
  s_b4a4x32kf_nb_sys2_vacc_hmc_vacc_miss_data_cnt_user_data_in : xbsIndex_r4/Gateway Out  inherit_from_input=off  hdl_port=on  rows=1  columns=1  UseAsDAC=off  DACChannel='1'  interface=None  automatic_assignment=on  address_offset=hex2dec('00')  intf_name=''  intf_description=''  timing_constraint=None  locs_specified=off  LOCs={}  io_standard={}  block_type=gatewayout
      settings: SourceProductName=The database /home/jmanley/.matlab/R2018a/slblocks_master.db is locked, or a table in the database is locked. (database is locked)
  sim_out : Terminator
  wires:
  io_delay/1 -> cast_gw/1
  cast_gw/1 -> s_b4a4x32kf_nb_sys2_vacc_hmc_vacc_miss_data_cnt_user_data_in/1
  s_b4a4x32kf_nb_sys2_vacc_hmc_vacc_miss_data_cnt_user_data_in/1 -> sim_out/1
  out_reg/1 -> assert_reg/1
  assert_reg/1 -> reint1/1
  reint1/1 -> io_delay/1

== system s_b4a4x32kf_nb/sys2/vacc/hmc_vacc/reord_miss_cnt ==
  out_reg : Inport
  assert_reg : xbsIndex_r4/Assert  assert_type=on  type_source=Explicitly  gui_display_data_type=Fixed-point  arith_type=Unsigned  n_bits=32  bin_pt=0  preci_type=Single  exp_width=8  frac_width=24  assert_rate=off  rate_source=Explicitly  period=1  output_port=on  block_type=assert
      settings: SourceProductName=The database /home/jmanley/.matlab/R2018a/slblocks_master.db is locked, or a table in the database is locked. (database is locked)
  cast_gw : xbsIndex_r4/Convert  gui_display_data_type=Fixed-point  arith_type=Unsigned  n_bits=32  bin_pt=0  float_type=Single  exp_bits=8  fraction_bits=24  quantization=Truncate  overflow=Wrap  en=off  latency=1  pipeline=off  dbl_ovrd=off  block_type=convert
      settings: SourceProductName=The database /home/jmanley/.matlab/R2018a/slblocks_master.db is locked, or a table in the database is locked. (database is locked)
  io_delay : xbsIndex_r4/Delay  rst=off  infoeditControl=Selection of Reset will increase slice count due to use of real FFs and instead of SRLs  en=off  latency=0  reg_retiming=on  dbl_ovrd=off  block_type=delay
      settings: SourceProductName=The database /home/jmanley/.matlab/R2018a/slblocks_master.db is locked, or a table in the database is locked. (database is locked)
  reint1 : xbsIndex_r4/Reinterpret  force_arith_type=on  arith_type=Unsigned  force_bin_pt=on  bin_pt=0  block_type=reinterpret
      settings: SourceProductName=The database /home/jmanley/.matlab/R2018a/slblocks_master.db is locked, or a table in the database is locked. (database is locked)
  s_b4a4x32kf_nb_sys2_vacc_hmc_vacc_reord_miss_cnt_user_data_in : xbsIndex_r4/Gateway Out  inherit_from_input=off  hdl_port=on  rows=1  columns=1  UseAsDAC=off  DACChannel='1'  interface=None  automatic_assignment=on  address_offset=hex2dec('00')  intf_name=''  intf_description=''  timing_constraint=None  locs_specified=off  LOCs={}  io_standard={}  block_type=gatewayout
      settings: SourceProductName=The database /home/jmanley/.matlab/R2018a/slblocks_master.db is locked, or a table in the database is locked. (database is locked)
  sim_out : Terminator
  wires:
  io_delay/1 -> cast_gw/1
  cast_gw/1 -> s_b4a4x32kf_nb_sys2_vacc_hmc_vacc_reord_miss_cnt_user_data_in/1
  s_b4a4x32kf_nb_sys2_vacc_hmc_vacc_reord_miss_cnt_user_data_in/1 -> sim_out/1
  out_reg/1 -> assert_reg/1
  assert_reg/1 -> reint1/1
  reint1/1 -> io_delay/1

== system s_b4a4x32kf_nb/sys2/vacc/hmc_vacc/reord_out_cnt ==
  out_reg : Inport
  assert_reg : xbsIndex_r4/Assert  assert_type=on  type_source=Explicitly  gui_display_data_type=Fixed-point  arith_type=Unsigned  n_bits=32  bin_pt=0  preci_type=Single  exp_width=8  frac_width=24  assert_rate=off  rate_source=Explicitly  period=1  output_port=on  block_type=assert
      settings: SourceProductName=The database /home/jmanley/.matlab/R2018a/slblocks_master.db is locked, or a table in the database is locked. (database is locked)
  cast_gw : xbsIndex_r4/Convert  gui_display_data_type=Fixed-point  arith_type=Unsigned  n_bits=32  bin_pt=0  float_type=Single  exp_bits=8  fraction_bits=24  quantization=Truncate  overflow=Wrap  en=off  latency=1  pipeline=off  dbl_ovrd=off  block_type=convert
      settings: SourceProductName=The database /home/jmanley/.matlab/R2018a/slblocks_master.db is locked, or a table in the database is locked. (database is locked)
  io_delay : xbsIndex_r4/Delay  rst=off  infoeditControl=Selection of Reset will increase slice count due to use of real FFs and instead of SRLs  en=off  latency=0  reg_retiming=on  dbl_ovrd=off  block_type=delay
      settings: SourceProductName=The database /home/jmanley/.matlab/R2018a/slblocks_master.db is locked, or a table in the database is locked. (database is locked)
  reint1 : xbsIndex_r4/Reinterpret  force_arith_type=on  arith_type=Unsigned  force_bin_pt=on  bin_pt=0  block_type=reinterpret
      settings: SourceProductName=The database /home/jmanley/.matlab/R2018a/slblocks_master.db is locked, or a table in the database is locked. (database is locked)
  s_b4a4x32kf_nb_sys2_vacc_hmc_vacc_reord_out_cnt_user_data_in : xbsIndex_r4/Gateway Out  inherit_from_input=off  hdl_port=on  rows=1  columns=1  UseAsDAC=off  DACChannel='1'  interface=None  automatic_assignment=on  address_offset=hex2dec('00')  intf_name=''  intf_description=''  timing_constraint=None  locs_specified=off  LOCs={}  io_standard={}  block_type=gatewayout
      settings: SourceProductName=The database /home/jmanley/.matlab/R2018a/slblocks_master.db is locked, or a table in the database is locked. (database is locked)
  sim_out : Terminator
  wires:
  io_delay/1 -> cast_gw/1
  cast_gw/1 -> s_b4a4x32kf_nb_sys2_vacc_hmc_vacc_reord_out_cnt_user_data_in/1
  s_b4a4x32kf_nb_sys2_vacc_hmc_vacc_reord_out_cnt_user_data_in/1 -> sim_out/1
  out_reg/1 -> assert_reg/1
  assert_reg/1 -> reint1/1
  reint1/1 -> io_delay/1
